simulink model "boost_openloop_models"  (R2025a)
settings: Solver=ode23tb  StartTime=0.0  StopTime=0.5  MaxStep=5e-06  RelTol=1e-05
PreLoadFcn:
  | if ~exist('BM', 'var'), boost_mrac_params; end
InitFcn:
  | if ~exist('BM', 'var'), boost_mrac_params; end
undefined symbols (not defined in the file): BM
libraries: spsSeriesRLCBranchLib x5, spsIdealSwitchLib x2, simulink x1, spsDiodeLib x1, spsMosfetLib x1, spsControlledVoltageSourceLib x1, spsCurrentMeasurementLib x1, spsVoltageMeasurementLib x1, sps_lib x1
Description:
  | Open-loop comparison of the model types of Section III (Fig. 7), Yanarates & Zhou (2022).
settings Model: Creator=runner  LastModifiedBy=runner
settings DataIOCC: SaveOutput=off  SignalLogging=off  SaveTime=off
settings DebuggingCC: AlgebraicLoopMsg=error

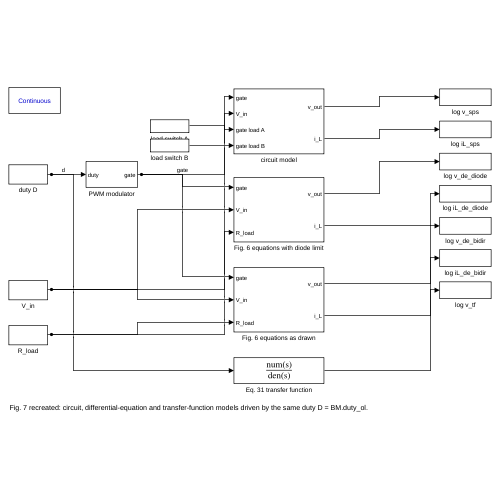
[thumbnail: Simulink's stored preview of the top-level diagram]
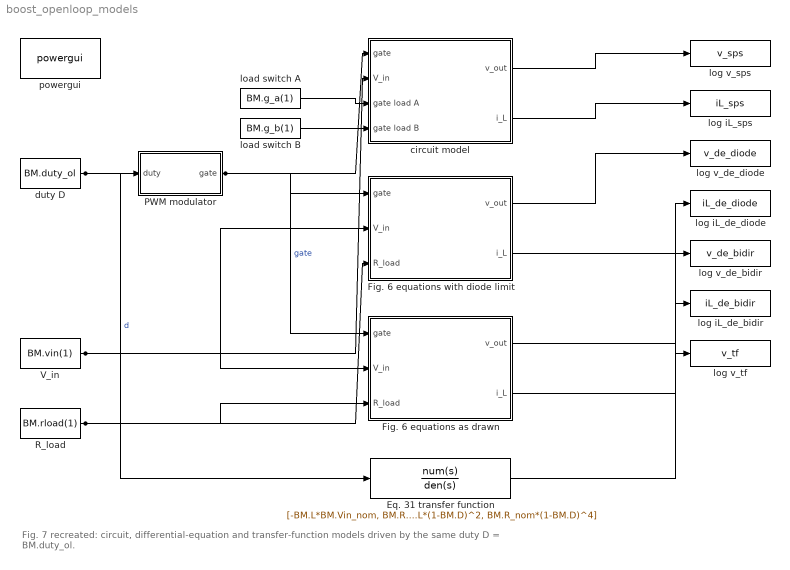
== system boost_openloop_models ==
  note: Fig. 7 recreated: circuit, differential-equation and transfer-function models driven by the same duty D = BM.duty_ol.
  Eq. 31 transfer function : TransferFcn  Numerator=[-BM.L*BM.Vin_nom, BM.R_nom*BM.Vin_nom*(1-BM.D)^2]  Denominator=[BM.L*BM.R_nom*BM.C*(1-BM.D)^2, BM.L*(1-BM.D)^2, BM.R_nom*(1-BM.D)^4]
  Fig. 6 equations as drawn : Subsystem
  Fig. 6 equations with diode limit : Subsystem
  PWM modulator : Subsystem
  R_load : Constant  Value=BM.rload(1)
  V_in : Constant  Value=BM.vin(1)
  circuit model : Subsystem
  duty D : Constant  Value=BM.duty_ol
  load switch A : Constant  Value=BM.g_a(1)
  load switch B : Constant  Value=BM.g_b(1)
  log iL_de_bidir : ToWorkspace  VariableName=iL_de_bidir  SaveFormat=Timeseries  SampleTime=BM.Ts
  log iL_de_diode : ToWorkspace  VariableName=iL_de_diode  SaveFormat=Timeseries  SampleTime=BM.Ts
  log iL_sps : ToWorkspace  VariableName=iL_sps  SaveFormat=Timeseries  SampleTime=BM.Ts
  log v_de_bidir : ToWorkspace  VariableName=v_de_bidir  SaveFormat=Timeseries  SampleTime=BM.Ts
  log v_de_diode : ToWorkspace  VariableName=v_de_diode  SaveFormat=Timeseries  SampleTime=BM.Ts
  log v_sps : ToWorkspace  VariableName=v_sps  SaveFormat=Timeseries  SampleTime=BM.Ts
  log v_tf : ToWorkspace  VariableName=v_tf  SaveFormat=Timeseries  SampleTime=BM.Ts
  powergui : sps_lib/powergui  Priority=1  SimulationMode=Continuous  SampleTime=50e-6  frequency=60  Iterations=50  frequencyindice=0  Pbase=100e6  ErrMax=1e-4  UnitsV=kV  UnitsW=MW  buscounter=0  FunctionMessages=off  echomessages=off  EnableUseOfTLC=off  CurrentSourceSwitches=off  DisableSnubberDevices=off  DisableRonSwitches=off  DisableVfSwitches=off  DisplayEquations=off  AutomaticDiscreteSolvers=off  SolverType=Tustin/Backward Euler (TBE)  Interpol=off  ExternalGateDelay=off  methode=off  Ts=100  x0status=blocks  SPID=on  SwTol=0  HookPort=off  NonlinearTolerance=1e-4  nMaxIteration=100  ContinueOnMaxIteration=off  RestoreLinks=warning  ResistiveCurrentMeasurement=off  Frange=[0:2:500]  Ylog=off  Xlog=on  ShowGrid=off  save=off  variable=ZData  structure=0  ZoomFFT=off  StartTime=0.0  cycles=1  DisplayStyle=1  fundamental=60  FreqAxis=off  MaxFrequency=1000  frequencyindicesteady=1  RmsSteady=1  display=off
  wires:
  duty D/1 -> PWM modulator/1(duty), Eq. 31 transfer function/1  "d"
  PWM modulator/1(gate) -> circuit model/1(gate), Fig. 6 equations with diode limit/1(gate), Fig. 6 equations as drawn/1(gate)  "gate"
  V_in/1 -> circuit model/2(V_in), Fig. 6 equations with diode limit/2(V_in), Fig. 6 equations as drawn/2(V_in)
  load switch A/1 -> circuit model/3(gate load A)
  load switch B/1 -> circuit model/4(gate load B)
  R_load/1 -> Fig. 6 equations with diode limit/3(R_load), Fig. 6 equations as drawn/3(R_load)
  circuit model/1(v_out) -> log v_sps/1
  circuit model/2(i_L) -> log iL_sps/1
  Fig. 6 equations with diode limit/1(v_out) -> log v_de_diode/1
  Fig. 6 equations with diode limit/2(i_L) -> log iL_de_diode/1
  Fig. 6 equations as drawn/1(v_out) -> log v_de_bidir/1
  Fig. 6 equations as drawn/2(i_L) -> log iL_de_bidir/1
  Eq. 31 transfer function/1 -> log v_tf/1

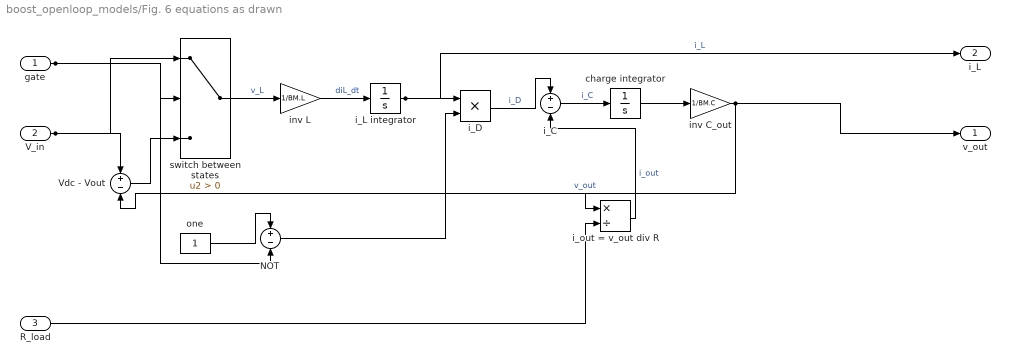
== system boost_openloop_models/Fig. 6 equations as drawn ==
  gate : Inport
  V_in : Inport  Port=2
  R_load : Inport  Port=3
  NOT : Sum  Inputs=+-
  Vdc - Vout : Sum  Inputs=+-
  charge integrator : Integrator  InitialCondition=BM.C*BM.v0
  i_C : Sum  Inputs=+-
  i_D : Product  Inputs=**
  i_L integrator : Integrator  InitialCondition=BM.iL0  LimitOutput=on  LowerSaturationLimit=-Inf
  i_out = v_out div R : Product  Inputs=*/
  inv C_out : Gain  Gain=1/BM.C
  inv L : Gain  Gain=1/BM.L
  one : Constant
  switch between states : Switch  Criteria=u2 > Threshold  SaturateOnIntegerOverflow=off  InputSameDT=off
  v_out : Outport
  i_L : Outport  Port=2
  wires:
  V_in/1 -> switch between states/1, Vdc - Vout/1
  gate/1 -> switch between states/2, NOT/2
  Vdc - Vout/1 -> switch between states/3
  switch between states/1 -> inv L/1  "v_L"
  inv L/1 -> i_L integrator/1  "diL_dt"
  i_L integrator/1 -> i_D/1, i_L/1  "i_L"
  one/1 -> NOT/1
  NOT/1 -> i_D/2
  i_D/1 -> i_C/1  "i_D"
  i_out = v_out div R/1 -> i_C/2  "i_out"
  i_C/1 -> charge integrator/1  "i_C"
  charge integrator/1 -> inv C_out/1
  inv C_out/1 -> v_out/1, Vdc - Vout/2, i_out = v_out div R/1  "v_out"
  R_load/1 -> i_out = v_out div R/2

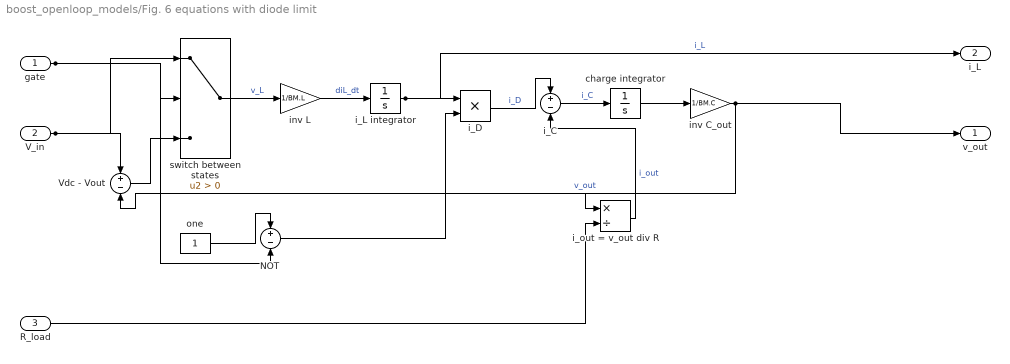
== system boost_openloop_models/Fig. 6 equations with diode limit ==
  gate : Inport
  V_in : Inport  Port=2
  R_load : Inport  Port=3
  NOT : Sum  Inputs=+-
  Vdc - Vout : Sum  Inputs=+-
  charge integrator : Integrator  InitialCondition=BM.C*BM.v0
  i_C : Sum  Inputs=+-
  i_D : Product  Inputs=**
  i_L integrator : Integrator  InitialCondition=BM.iL0  LimitOutput=on  LowerSaturationLimit=BM.iL_min
  i_out = v_out div R : Product  Inputs=*/
  inv C_out : Gain  Gain=1/BM.C
  inv L : Gain  Gain=1/BM.L
  one : Constant
  switch between states : Switch  Criteria=u2 > Threshold  SaturateOnIntegerOverflow=off  InputSameDT=off
  v_out : Outport
  i_L : Outport  Port=2
  wires:
  V_in/1 -> switch between states/1, Vdc - Vout/1
  gate/1 -> switch between states/2, NOT/2
  Vdc - Vout/1 -> switch between states/3
  switch between states/1 -> inv L/1  "v_L"
  inv L/1 -> i_L integrator/1  "diL_dt"
  i_L integrator/1 -> i_D/1, i_L/1  "i_L"
  one/1 -> NOT/1
  NOT/1 -> i_D/2
  i_D/1 -> i_C/1  "i_D"
  i_out = v_out div R/1 -> i_C/2  "i_out"
  i_C/1 -> charge integrator/1  "i_C"
  charge integrator/1 -> inv C_out/1
  inv C_out/1 -> v_out/1, Vdc - Vout/2, i_out = v_out div R/1  "v_out"
  R_load/1 -> i_out = v_out div R/2

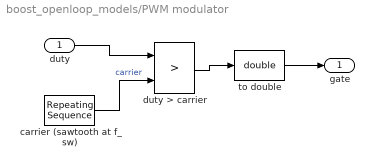
== system boost_openloop_models/PWM modulator ==
  duty : Inport
  carrier (sawtooth at f_sw) : simulink/Sources/Repeating Sequence  rep_seq_t=[0 BM.Tsw]  rep_seq_y=[0 1]
  duty > carrier : RelationalOperator  Operator=>  OutDataTypeStr=boolean  RndMeth=Simplest  InputSameDT=off
  to double : DataTypeConversion  OutDataTypeStr=double  SaturateOnIntegerOverflow=off  RndMeth=Floor
  gate : Outport
  wires:
  duty/1 -> duty > carrier/1
  carrier (sawtooth at f_sw)/1 -> duty > carrier/2  "carrier"
  duty > carrier/1 -> to double/1
  to double/1 -> gate/1

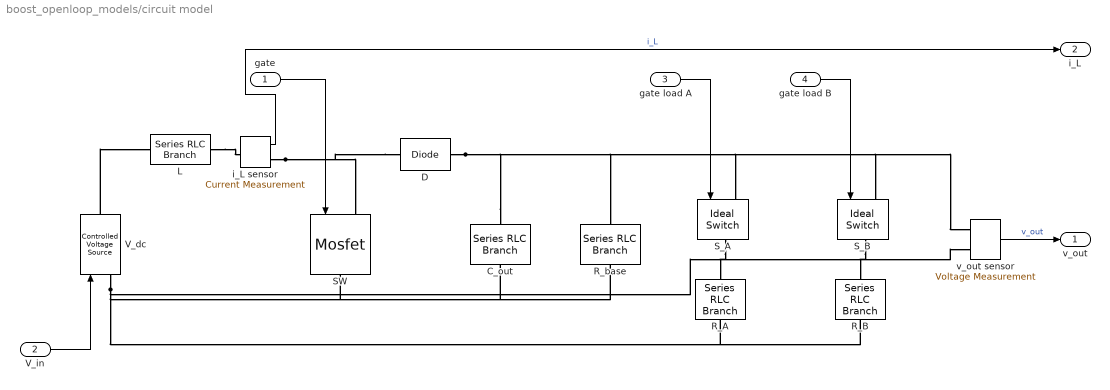
== system boost_openloop_models/circuit model ==
  gate : Inport
  V_in : Inport  Port=2
  gate load A : Inport  Port=3
  gate load B : Inport  Port=4
  C_out : spsSeriesRLCBranchLib/Series RLC Branch  LConnTagsString=__new0  RConnTagsString=__new0  BranchType=C  Resistance=1  Inductance=1e-3  SetiL0=off  InitialCurrent=0  Capacitance=BM.C  Setx0=on  InitialVoltage=BM.v0  Measurements=None
  D : spsDiodeLib/Diode  Ron=BM.Ron_d  Lon=0  Vf=BM.Vf_d  IC=0  UseSnubber=0  Rs=inf  Cs=0  Measurements=off
  L : spsSeriesRLCBranchLib/Series RLC Branch  LConnTagsString=__new0  RConnTagsString=__new0  BranchType=L  Resistance=1  Inductance=BM.L  SetiL0=on  InitialCurrent=BM.iL0  Capacitance=1e-6  Setx0=off  InitialVoltage=0  Measurements=None
  R_A : spsSeriesRLCBranchLib/Series RLC Branch  LConnTagsString=__new0  RConnTagsString=__new0  BranchType=R  Resistance=BM.R_a  Inductance=1e-3  SetiL0=off  InitialCurrent=0  Capacitance=1e-6  Setx0=off  InitialVoltage=0  Measurements=None
  R_B : spsSeriesRLCBranchLib/Series RLC Branch  LConnTagsString=__new0  RConnTagsString=__new0  BranchType=R  Resistance=BM.R_b  Inductance=1e-3  SetiL0=off  InitialCurrent=0  Capacitance=1e-6  Setx0=off  InitialVoltage=0  Measurements=None
  R_base : spsSeriesRLCBranchLib/Series RLC Branch  LConnTagsString=__new0  RConnTagsString=__new0  BranchType=R  Resistance=BM.R_base  Inductance=1e-3  SetiL0=off  InitialCurrent=0  Capacitance=1e-6  Setx0=off  InitialVoltage=0  Measurements=None
  SW : spsMosfetLib/Mosfet  Ron=BM.Ron_sw  Lon=0  Rd=0.01  Vfd=0  IC=0  Rs=1e5  Cs=inf  Measurements=off
  S_A : spsIdealSwitchLib/Ideal Switch  Ron=1e-3  Lon=0  IC=0  Rs=1e5  Cs=inf  Measurements=off
  S_B : spsIdealSwitchLib/Ideal Switch  Ron=1e-3  Lon=0  IC=0  Rs=1e5  Cs=inf  Measurements=off
  V_dc : spsControlledVoltageSourceLib/Controlled Voltage Source  Initialize=on  Source_Type=DC  Amplitude=BM.vin(1)  Phase=0  Frequency=0  Measurements=None
  i_L sensor : spsCurrentMeasurementLib/Current Measurement  PhasorSimulation=off  OutputType=Complex  PSBequivalent=0
  v_out sensor : spsVoltageMeasurementLib/Voltage Measurement  PhasorSimulation=off  OutputType=Complex  PSBequivalent=0
  v_out : Outport
  i_L : Outport  Port=2
  wires:
  V_in/1 -> V_dc/1
  gate/1 -> SW/1
  gate load A/1 -> S_A/1
  gate load B/1 -> S_B/1
  i_L sensor/1 -> i_L/1  "i_L"
  v_out sensor/1 -> v_out/1  "v_out"
  connections:
  V_dc/RConn1 -- L/LConn1
  L/RConn1 -- i_L sensor/LConn1
  D/LConn1 -- i_L sensor/RConn1 -- SW/LConn1
  C_out/LConn1 -- D/RConn1 -- R_base/LConn1 -- S_A/LConn1 -- S_B/LConn1 -- v_out sensor/LConn1
  S_A/RConn1 -- R_A/LConn1
  S_B/RConn1 -- R_B/LConn1
  SW/RConn1 -- V_dc/LConn1 -- C_out/RConn1 -- R_base/RConn1 -- R_A/RConn1 -- R_B/RConn1 -- v_out sensor/LConn2
